simulink model "day1_dc_motor_open_loop"  (R2026a)
settings: Solver=VariableStepAuto  StopTime=2.0
undefined symbols (not defined in the file): b, J, Ke, Kt, L, R, rad_to_rpm, T_load, V_test
settings Model: Creator=DELL  LastModifiedBy=DELL

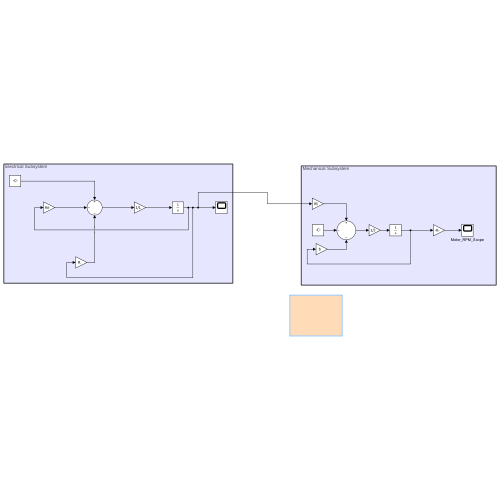
[thumbnail: Simulink's stored preview of the top-level diagram]
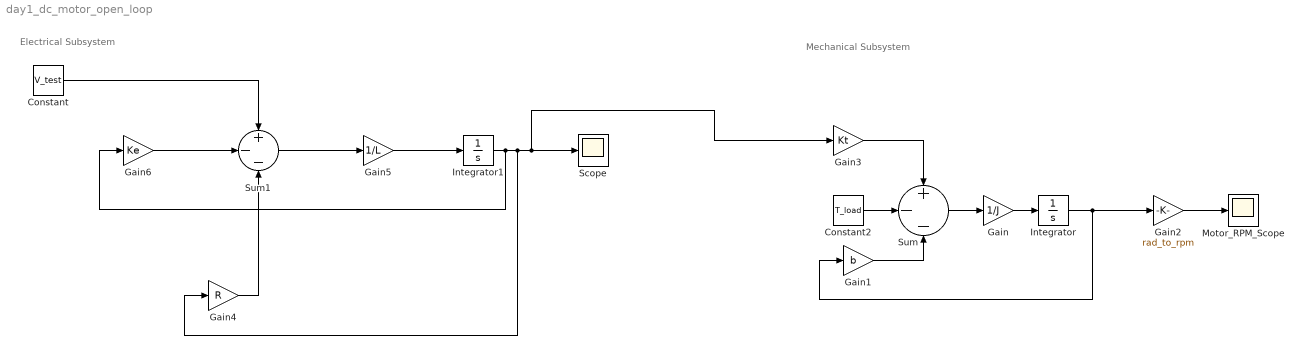
== system day1_dc_motor_open_loop ==
  note: Electrical Subsystem
  note: Mechanical Subsystem
  Constant : Constant  Value=V_test
  Constant2 : Constant  Value=T_load
  Gain : Gain  Gain=1/J
  Gain1 : Gain  Gain=b
  Gain2 : Gain  Gain=rad_to_rpm
  Gain3 : Gain  Gain=Kt
  Gain4 : Gain  Gain=R
  Gain5 : Gain  Gain=1/L
  Gain6 : Gain  Gain=Ke
  Integrator : Integrator
  Integrator1 : Integrator
  Motor_RPM_Scope : Scope
      settings: ActiveDisplayYMinimum=-5469.5785327149169  ActiveDisplayYMaximum=41734.903297781719
  Scope : Scope
      settings: ActiveDisplayYMinimum=-0.046366756718675572  ActiveDisplayYMaximum=4.9531791851211349
  Sum : Sum  Inputs=+--
  Sum1 : Sum  Inputs=+--
  wires:
  Gain3/1 -> Sum/1
  Gain/1 -> Integrator/1
  Constant2/1 -> Sum/2
  Gain1/1 -> Sum/3
  Gain2/1 -> Motor_RPM_Scope/1
  Sum/1 -> Gain/1
  Integrator/1 -> Gain1/1, Gain2/1
  Integrator1/1 -> Gain6/1, Gain4/1, Gain3/1, Scope/1
  Gain4/1 -> Sum1/3
  Gain5/1 -> Integrator1/1
  Gain6/1 -> Sum1/2
  Constant/1 -> Sum1/1
  Sum1/1 -> Gain5/1
